simulink model "nonLinearPlant2024"  (R2024a)
settings: Solver=ode45  StartTime=0.0  StopTime=10  RelTol=1e-3
undefined symbols (not defined in the file or in its folder): fractalcoef
libraries: instrumentseriallib x3, simulink x2, instrumentlib x2, mspfiltlib x1, mspsensorlib x1, simulink_extras x1, slpidlib x1
settings Model: LastModifiedBy=saman
settings SolverCC: AutoInsertRateTranBlk=on
settings OptimizationCC: DefaultParameterBehavior=Inlined  EnhancedBackFolding=on  PassReuseOutputArgsAs=Individual arguments  ZeroExternalMemoryAtStartup=off  ZeroInternalMemoryAtStartup=off  MaxStackSize=64  OptimizeBlockOrder=speed  DifferentSizesBufferReuse=on  EfficientTunableParamExpr=on
settings DebuggingCC: ParameterTunabilityLossMsg=error
settings HardwareCC: ProdBitPerPointer=32  ProdBitPerSizeT=32  ProdBitPerPtrDiffT=32  ProdLargestAtomicInteger=Long  ProdLargestAtomicFloat=Double  ProdWordSize=32  ProdHWDeviceType=ARM Compatible->ARM Cortex  UseEmbeddedCoderFeatures=off  UseSimulinkCoderFeatures=off
settings ModelReferenceCC: UpdateModelReferenceTargets=IfOutOfDate
settings SFSimCC: MATLABDynamicMemAlloc=off
settings RTWCC: Description=Embedded Coder  SystemTargetFile=ert.tlc  TemplateMakefile=ert_default_tmf  Toolchain=Arduino ARM  BuildConfiguration=Faster Runs
settings CodeAppCC: ForceParamTrailComments=on  IgnoreCustomStorageClasses=off  OperatorAnnotations=on  SimulinkDataObjDesc=on  SFDataObjDesc=on  InsertBlockDesc=on
settings ERTTargetCC: SupportContinuousTime=on  SupportNonInlinedSFcns=on  ExtModeTransport=3  ExtModeStaticAlloc=on  ExtModeStaticAllocSize=24576  ExtModeMexFile=ext_xcp  ExtModeIntrfLevel=Level2 - Open  InlinedParameterPlacement=NonHierarchical  ERTCustomFileTemplate=example_file_process.tlc

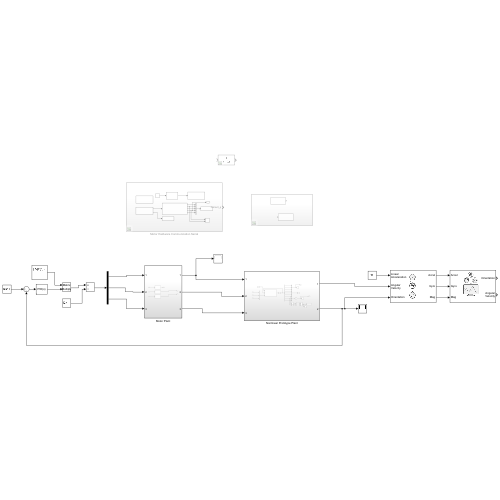
[thumbnail: Simulink's stored preview of the top-level diagram]
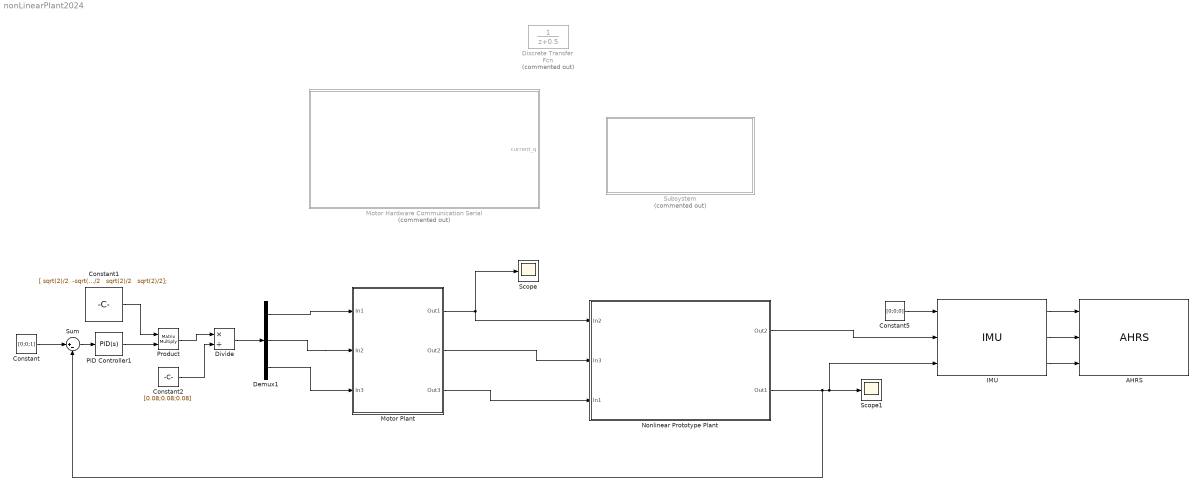
== system nonLinearPlant2024 ==
  AHRS : mspfiltlib/AHRS  DispRefFrame=ENU  DecimationFactor=1  InitialProcessNoise=ahrsfilter.defaultProcessNoise  OrientationFormat=quaternion  SimulateUsing=Interpreted execution  AccelerometerNoise=0.0001924722  GyroscopeNoise=9.1385e-5  MagnetometerNoise=0.1  GyroscopeDriftNoise=3.0462e-13  LinearAccelerationNoise=0.0096236100000000012  MagneticDisturbanceNoise=0.5  LinearAccelerationDecayFactor=0.5  MagneticDisturbanceDecayFactor=0.5  ExpectedMagneticFieldStrength=50
  Constant : Constant  Value=[0;0;1]
  Constant1 : Constant  Value=|
      | [ sqrt(2)/2  -sqrt(2)/4  -sqrt(2)/4;
      |                0           sqrt(6)/4  -sqrt(6)/4;
      |                sqrt(2)/2   sqrt(2)/2   sqrt(2)/2];
  Constant2 : Constant  Value=[0.08;0.08;0.08]
  Constant5 : Constant  Value=[0;0;0]
  Demux1 : Demux  Outputs=3
  Discrete Transfer Fcn : DiscreteTransferFcn  Commented=on
  Divide : Product  Inputs=*/
  IMU : mspsensorlib/IMU  DispRefFrame=ENU  TemperaturePort=off  Temperature=25  MagneticFieldPort=off  MagneticFieldNED=[ 27.5550, -2.4169, -16.0849 ]  MagneticFieldENU=[ -2.4169, 27.5550, 16.0849 ]  SeedDouble=67  SimulateUsing=Interpreted execution  AccelParamsMeasurementRange=Inf  AccelParamsResolution=0  AccelParamsConstantBias=[ 0, 0, 0 ]  AccelParamsAxesMisalignment=[ 100, 0, 0; 0, 100, 0; 0, 0, 100 ]  AccelParamsNoiseDensity=[ 0, 0, 0 ]  AccelParamsBiasInstability=[ 0, 0, 0 ]  AccelParamsBiasInstabilityNumerator=fractalcoef().Numerator  AccelParamsBiasInstabilityDenominator=fractalcoef().Denominator  AccelParamsRandomWalk=[ 0, 0, 0 ]  AccelParamsNoiseType=double-sided  AccelParamsTemperatureBias=[ 0, 0, 0 ]  AccelParamsTemperatureScaleFactor=[ 0, 0, 0 ]  GyroParamsMeasurementRange=Inf  GyroParamsResolution=0  GyroParamsConstantBias=[ 0, 0, 0 ]  GyroParamsAxesMisalignment=[ 100, 0, 0; 0, 100, 0; 0, 0, 100 ]  GyroParamsAccelerationBias=[ 0, 0, 0 ]  GyroParamsNoiseDensity=[ 0, 0, 0 ]  GyroParamsBiasInstability=[ 0, 0, 0 ]  GyroParamsBiasInstabilityNumerator=fractalcoef().Numerator  GyroParamsBiasInstabilityDenominator=fractalcoef().Denominator  GyroParamsRandomWalk=[ 0, 0, 0 ]  GyroParamsNoiseType=double-sided  GyroParamsTemperatureBias=[ 0, 0, 0 ]  GyroParamsTemperatureScaleFactor=[ 0, 0, 0 ]  MagParamsMeasurementRange=Inf  MagParamsResolution=0  MagParamsConstantBias=[ 0, 0, 0 ]  MagParamsAxesMisalignment=[ 100, 0, 0; 0, 100, 0; 0, 0, 100 ]  MagParamsNoiseDensity=[ 0, 0, 0 ]  MagParamsBiasInstability=[ 0, 0, 0 ]  MagParamsBiasInstabilityNumerator=fractalcoef().Numerator  MagParamsBiasInstabilityDenominator=fractalcoef().Denominator  MagParamsRandomWalk=[ 0, 0, 0 ]  MagParamsNoiseType=double-sided  MagParamsTemperatureBias=[ 0, 0, 0 ]  MagParamsTemperatureScaleFactor=[ 0, 0, 0 ]
  Motor Hardware Communication Serial : Subsystem  Commented=on
  Motor Plant : Subsystem
  Nonlinear Prototype Plant : Subsystem
  PID Controller1 : slpidlib/PID Controller  Controller=PID  Form=Parallel  TimeDomain=Continuous-time  UseExternalTs=off  SampleTime=-1  IntegratorMethod=Forward Euler  FilterMethod=Forward Euler  ControllerParametersSource=internal  P=1  I=1  UseKiTs=off  D=0  UseExternalDerivativeSource=off  N=100  UseFilter=on  TunerSelectOption=Transfer Function Based (PID Tuner App)  InitialConditionSource=internal  InitialConditionForIntegrator=0  InitialConditionForFilter=0  DifferentiatorICPrevScaledInput=0  ExternalReset=none  TrackingMode=off  Kt=1  LimitOutput=off  SatLimitsSource=internal  UpperSaturationLimit=inf  LowerSaturationLimit=-inf  LinearizeAsGain=on  AntiWindupMode=none  Kb=1  LimitIntegrator=off  UpperIntegratorSaturationLimit=inf  LowerIntegratorSaturationLimit=-inf  POutMin=[]  POutMax=[]  IOutMin=[]  IOutMax=[]  DOutMin=[]  DOutMax=[]  NOutMin=[]  NOutMax=[]  SumOutMin=[]  SumOutMax=[]  SaturationOutMin=[]  SaturationOutMax=[]  PParamMin=[]  PParamMax=[]  IParamMin=[]  IParamMax=[]  DParamMin=[]  DParamMax=[]  NParamMin=[]  NParamMax=[]  KbParamMin=[]  KbParamMax=[]  KtParamMin=[]  KtParamMax=[]  KbOutMin=[]  KbOutMax=[]  KtOutMin=[]  KtOutMax=[]  IntegratorOutMin=[]  IntegratorOutMax=[]  FilterOutMin=[]  FilterOutMax=[]  SumI1OutMin=[]  SumI1OutMax=[]  SumI2OutMin=[]  SumI2OutMax=[]  SumI3OutMin=[]  SumI3OutMax=[]  SumI4OutMin=[]  SumI4OutMax=[]  SumDOutMin=[]  SumDOutMax=[]  DifferentiatorOutMin=[]  DifferentiatorOutMax=[]  FilterDiffOutCoefMin=[]  FilterDiffOutCoefMax=[]  ReciprocalOutMin=[]  ReciprocalOutMax=[]  SumDenOutMin=[]  SumDenOutMax=[]  SumNumOutMin=[]  SumNumOutMax=[]  DivideOutMin=[]  DivideOutMax=[]  UdiffTsProdOutMin=[]  UdiffTsProdOutMax=[]  NTsProdOutMin=[]  NTsProdOutMax=[]  UintegralTsProdOutMin=[]  UintegralTsProdOutMax=[]  UngainTsProdOutMin=[]  UngainTsProdOutMax=[]  ClampingZeroOutDataTypeStr=Inherit: Inherit via back propagation  ClampingZeroOutMin=[]  ClampingZeroOutMax=[]  FilterDenConstantOutDataTypeStr=Inherit: Inherit via back propagation  FilterDenConstantOutMin=[]  FilterDenConstantOutMax=[]  PCopyOutDataTypeStr=Inherit: Inherit via back propagation  PCopyOutMin=[]  PCopyOutMax=[]  NCopyOutDataTypeStr=Inherit: Inherit via back propagation  NCopyOutMin=[]  NCopyOutMax=[]  IntegratorContinuousStateAttributes=''  IntegratorStateMustResolveToSignalObject=off  IntegratorRTWStateStorageClass=Auto  FilterContinuousStateAttributes=''  FilterStateMustResolveToSignalObject=off  FilterRTWStateStorageClass=Auto  ParallelPVariant=InternalParameters  IdealPVariant=Disabled  IVariant=InternalParameters  DVariant=InternalParameters  IntegratorVariant=Continuous  SatVariant=Disabled  AWVariant=Passthrough  PCopyVariant=Disabled  TRVariant=Disabled  FdbkBlocksVariant=Forward  IdealPFdbkVariant=Disabled  SatFdbkVariant=Disabled  DerivativeFilterVariant=ContFilter  NVariant=InternalParameters  NCopyVariant=Disabled  FilterICVariant=InternalICsFilter  IntegratorICVariant=InternalICs  ExternalResetVariant=Disabled  TRSumVariant=Passthrough  SumFdbkVariant=Disabled  SumVariant=Sum_PID  TsampFilterVariant=InternalTs  TsampNgainVariant=Passthrough  TsampIntegralVariant=Disabled_SignalSpec  ExternalSaturationOutDataTypeStr=Inherit: Same as second input  DerivativeSourceVariant=ErrorSignal
  Product : Product  Multiplication=Matrix(*)
  Scope : Scope
  Scope1 : Scope
  Subsystem : Subsystem  Commented=on
  Sum : Sum  Inputs=|+-
  wires:
  Nonlinear Prototype Plant/2(Out1) -> Sum/2, IMU/3, Scope1/1
  Constant/1 -> Sum/1
  Motor Plant/1(Out1) -> Scope/1, Nonlinear Prototype Plant/1(In2)
  Demux1/2 -> Motor Plant/2(In2)
  Demux1/3 -> Motor Plant/3(In3)
  Motor Plant/2(Out2) -> Nonlinear Prototype Plant/2(In3)
  Motor Plant/3(Out3) -> Nonlinear Prototype Plant/3(In1)
  Product/1 -> Divide/1
  Demux1/1 -> Motor Plant/1(In1)
  Constant1/1 -> Product/1
  Sum/1 -> PID Controller1/1
  PID Controller1/1 -> Product/2
  Divide/1 -> Demux1/1
  Constant2/1 -> Divide/2
  Nonlinear Prototype Plant/1(Out2) -> IMU/2
  Constant5/1 -> IMU/1
  IMU/1 -> AHRS/1
  IMU/2 -> AHRS/2
  IMU/3 -> AHRS/3

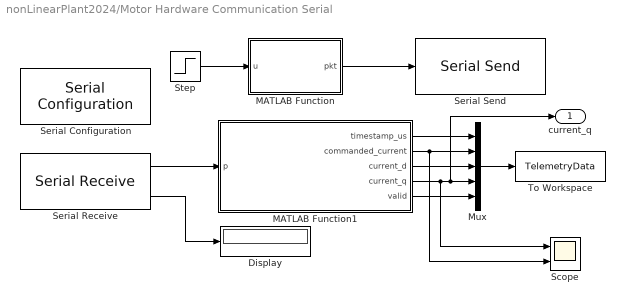
== system nonLinearPlant2024/Motor Hardware Communication Serial ==
  Display : Display
  MATLAB Function : MATLAB Function  TreatAsAtomicUnit=on
  MATLAB Function1 : MATLAB Function  TreatAsAtomicUnit=on
  Mux : Mux  Inputs=5
  Scope : Scope  NumInputPorts=2
  Serial Configuration : instrumentseriallib/Serial Configuration  Priority=-200000  PortSel=COM10  Port=COM10  ComPort=COM10  BaudRate=115200  DataBits=8  Parity=none  StopBits=1  ByteOrder=little-endian  FlowControl=none  Timeout=10  SimulateUsing=Interpreted execution  BlockInModel=on  aMode=1
  Serial Receive : instrumentseriallib/Serial Receive  Priority=1  PortSel=COM10  Port=COM10  ComPort=COM10  DataType=uint8  SaveDataType=uint8  ToggleHeader=on  Header=[165 90]  ToggleDataSize=on  DataSize=[17 1]  ToggleTerminator=on  Terminator=<none>  CustomTerminator=[]  InputFormat=Column major  EnableBlockingMode=off  ActionDataUnavailable=Output last received value  ActionWhenDataUnavailable=Output last received value  CustomValue=0  SampleTime=0.01  SimulateUsing=Interpreted execution  BlockInModel=on  aMode=1
  Serial Send : instrumentseriallib/Serial Send  Priority=1  PortSel=COM10  Port=COM10  ComPort=COM10  Header=[]  Terminator=<none>  CustomTerminator=[]  EnableBlockingMode=off  SimulateUsing=Interpreted execution  BlockInModel=on  aMode=1
  Step : Step  After=0.055  SampleTime=0
  To Workspace : ToWorkspace  VariableName=TelemetryData  SaveFormat=Timeseries  SampleTime=-1
  current_q : Outport
  wires:
  MATLAB Function/1(pkt) -> Serial Send/1
  Step/1 -> MATLAB Function/1(u)
  Serial Receive/1 -> MATLAB Function1/1(p)
  Serial Receive/2 -> Display/1
  MATLAB Function1/1(timestamp_us) -> Mux/1
  MATLAB Function1/2(commanded_current) -> Scope/2, Mux/2
  MATLAB Function1/3(current_d) -> Mux/3
  MATLAB Function1/4(current_q) -> Scope/1, current_q/1, Mux/4
  MATLAB Function1/5(valid) -> Mux/5
  Mux/1 -> To Workspace/1

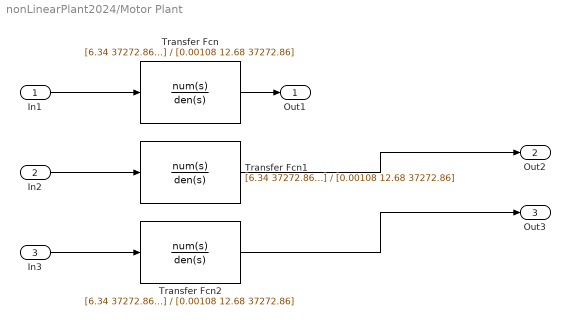
== system nonLinearPlant2024/Motor Plant ==
  In1 : Inport
  In2 : Inport  Port=2
  In3 : Inport  Port=3
  Transfer Fcn : TransferFcn  Numerator=[6.34 37272.86]  Denominator=[0.00108 12.68 37272.86]
  Transfer Fcn1 : TransferFcn  Numerator=[6.34 37272.86]  Denominator=[0.00108 12.68 37272.86]
  Transfer Fcn2 : TransferFcn  Numerator=[6.34 37272.86]  Denominator=[0.00108 12.68 37272.86]
  Out1 : Outport
  Out2 : Outport  Port=2
  Out3 : Outport  Port=3
  wires:
  In1/1 -> Transfer Fcn/1
  Transfer Fcn/1 -> Out1/1
  In3/1 -> Transfer Fcn2/1
  In2/1 -> Transfer Fcn1/1
  Transfer Fcn2/1 -> Out3/1
  Transfer Fcn1/1 -> Out2/1

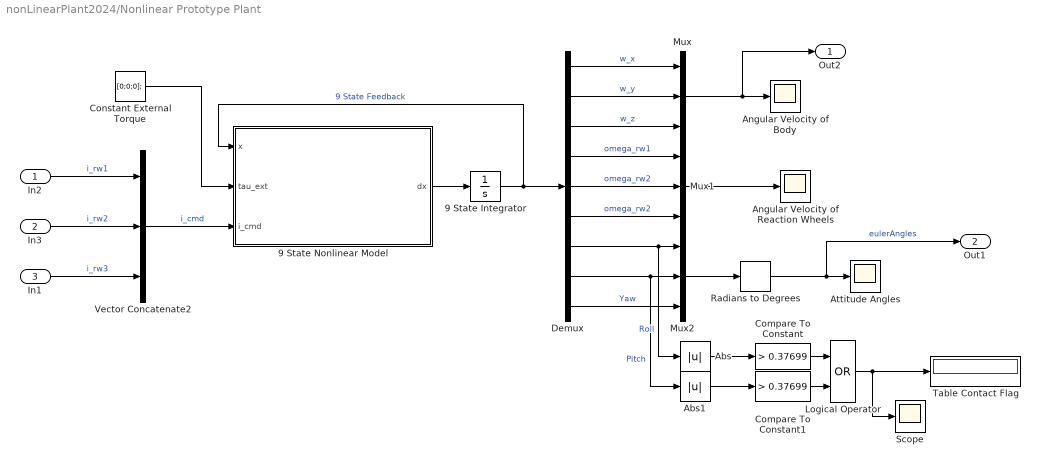
== system nonLinearPlant2024/Nonlinear Prototype Plant ==
  In2 : Inport
  In3 : Inport  Port=2
  In1 : Inport  Port=3
  9 State Integrator : Integrator  InitialCondition=zeros(9,1)  LimitOutput=on  UpperSaturationLimit=[Inf; Inf; Inf; 48.91; 48.91; 48.91; Inf; Inf; Inf];  LowerSaturationLimit=[-Inf; -Inf; -Inf; -48.91; -48.91; -48.91; -Inf; -Inf; -Inf];  ContinuousStateAttributes={'wX','wY','wZ','omegaX','omegaY','omegaZ','roll','pitch','yaw'}
  9 State Nonlinear Model : MATLAB Function  TreatAsAtomicUnit=on
  Abs : Abs  SaturateOnIntegerOverflow=off
  Abs1 : Abs  SaturateOnIntegerOverflow=off
  Angular Velocity of Body : Scope
  Angular Velocity of Reaction Wheels : Scope
  Attitude Angles : Scope
  Compare To Constant : simulink/Logic and Bit Operations/Compare To Constant  relop=>  const=0.37699  OutDataTypeStr=boolean
  Compare To Constant1 : simulink/Logic and Bit Operations/Compare To Constant  relop=>  const=0.37699  OutDataTypeStr=boolean
  Constant External Torque : Constant  Value=[0;0;0];
  Demux : Demux  Outputs=9
  Logical Operator : Logic  Operator=OR  AllPortsSameDT=off  OutDataTypeStr=boolean
  Mux : Mux  Inputs=3
  Mux1 : Mux  Inputs=3
  Mux2 : Mux  Inputs=3
  Radians to Degrees : simulink_extras/Transformations/Radians to Degrees
  Scope : Scope
  Table Contact Flag : Display
  Vector Concatenate2 : Concatenate  NumInputs=3
  Out2 : Outport
  Out1 : Outport  Port=2
  wires:
  Demux/5 -> Mux1/2  "omega_rw2"
  Compare To Constant/1 -> Logical Operator/1
  9 State Integrator/1 -> 9 State Nonlinear Model/1(x), Demux/1  "9 State Feedback"
  Demux/7 -> Abs/1, Mux2/1  "Roll"
  Demux/1 -> Mux/1  "w_x"
  Demux/4 -> Mux1/1  "omega_rw1"
  Demux/9 -> Mux2/3  "Yaw"
  Mux/1 -> Out2/1, Angular Velocity of Body/1
  Demux/3 -> Mux/3  "w_z"
  Constant External Torque/1 -> 9 State Nonlinear Model/2(tau_ext)
  Compare To Constant1/1 -> Logical Operator/2
  Demux/8 -> Abs1/1, Mux2/2  "Pitch"
  Abs1/1 -> Compare To Constant1/1
  Mux1/1 -> Angular Velocity of Reaction Wheels/1
  Demux/2 -> Mux/2  "w_y"
  Mux2/1 -> Radians to Degrees/1
  Abs/1 -> Compare To Constant/1
  9 State Nonlinear Model/1(dx) -> 9 State Integrator/1
  Vector Concatenate2/1 -> 9 State Nonlinear Model/3(i_cmd)  "i_cmd"
  Demux/6 -> Mux1/3  "omega_rw2"
  Radians to Degrees/1 -> Out1/1, Attitude Angles/1  "eulerAngles"
  Logical Operator/1 -> Scope/1, Table Contact Flag/1
  In1/1 -> Vector Concatenate2/3  "i_rw3"
  In3/1 -> Vector Concatenate2/2  "i_rw2"
  In2/1 -> Vector Concatenate2/1  "i_rw1"

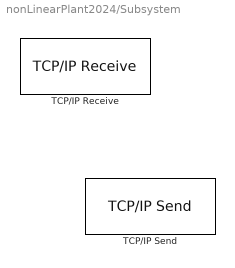
== system nonLinearPlant2024/Subsystem ==
  TCP/IP Receive : instrumentlib/TCP//IP Receive  Port=80  DataSize=[ 1, 1 ]  DataType=uint8  ASCIIFormatting=%f  Terminator=LF  CustomTerminator=10  ByteOrder=big-endian  EnableBlockingMode=on  Timeout=10  SampleTime=0.01  SimulateUsing=Interpreted execution
  TCP/IP Send : instrumentlib/TCP//IP Send  Port=80  ByteOrder=big-endian  EnableBlockingMode=on  Timeout=10  TransferDelay=on  SimulateUsing=Interpreted execution

== matlab function nonLinearPlant2024/Motor Hardware Communication Serial/MATLAB Function1 ==
  data: p input; timestamp_us output; commanded_current output; current_d output; current_q output; valid output
function [timestamp_us, commanded_current, current_d, current_q, valid] = UnpackTelemetry(p)
   
    % Input: 17 bytes after the A5 5A header
    % Payload: timestamp (uint32), commanded current, Id, Iq, checksum
    
    b = reshape(uint8(p), 1, 17);
    
    % Verify XOR checksum over timestamp and three current values
    cs = uint8(0);
    for k = 1:16
        cs = bitxor(cs, b(k));
    end
    
    valid = (cs == b(17));
    
    % Decode binary data
    timestamp_us = typecast(uint8(b(1:4)), 'uint32');
    commanded_current = typecast(uint8(b(5:8)), 'single');
    current_d = typecast(uint8(b(9:12)), 'single');
    current_q = typecast(uint8(b(13:16)), 'single');
    
    % Reject invalid current measurements
    if ~valid
        commanded_current = single(NaN);
        current_d = single(NaN);
        current_q = single(NaN);
    end
end

== matlab function nonLinearPlant2024/Motor Hardware Communication Serial/MATLAB Function ==
  data: u input; pkt output
function pkt = PackCommand(u)

    u = single(u);
    b = reshape(typecast(u, 'uint8'), 1, 4);
    
    pkt = zeros(1, 7, 'uint8');
    
    pkt(1) = uint8( hex2dec('A5') );
    pkt(2) = uint8( hex2dec('5A') );
    pkt(3:6) = b;
    
    cs = uint8(0);
    for k = 3:6
        cs = bitxor(cs, pkt(k));
    end
    
    pkt(7) = cs;
end

== matlab function nonLinearPlant2024/Nonlinear Prototype Plant/9 State Nonlinear Model ==
  data: x input; dx output; tau_ext input; i_cmd input
function dx = nonlinearPlant(x,tau_ext,i_cmd)
    
    % Protoype system inertia matrix
    I = [0.250909017 0 0;
         0 0.25037717 0;
         0 0 0.449674125];
    
    % RW inertia matrix
    I_rw = [0.000637038 0 0; 
            0 0.000637038 0;
            0 0 0.000637038];

    % Torque constant of rw, [Nm/A]
    kt_rw1 = 0.08; 
    kt_rw2 = 0.08;
    kt_rw3 = 0.08;

% Reaction wheel frame to body frame
    R_b_rw = [ sqrt(2)/2  -sqrt(2)/4  -sqrt(2)/4;
               0           sqrt(6)/4  -sqrt(6)/4;
               sqrt(2)/2   sqrt(2)/2   sqrt(2)/2];
    
    
    % Initiate states and vectors
    wx = x(1);
    wy = x(2);
    wz = x(3);
    
    Omega_x = x(4);
    Omega_y = x(5);
    Omega_z = x(6);
    
    phi   = x(7);
    theta = x(8);
    psi   = x(9);
    
    w = [wx;wy;wz];

    Omega = [Omega_x;Omega_y;Omega_z];

    % Reaction wheel input is current
    kt_rw = [kt_rw1;
             kt_rw2;
             kt_rw3];
 
    tau_rw = kt_rw .* i_cmd;

    Omega_dot = I_rw \ tau_rw;


    % Dynamic equation for prototype
    w_dot = I \ ( ...
        tau_ext ...
        - cross(w,I*w) ...
        - R_b_rw*(I_rw*Omega_dot) ...
        - cross(w,R_b_rw*(I_rw*Omega)) );

   % Euler kinematics
    phi_dot = ...
        wx ...
        + wy*sin(phi)*tan(theta) ...
        + wz*cos(phi)*tan(theta);
    
    theta_dot = ...
        wy*cos(phi) ...
        - wz*sin(phi);
    
    psi_dot = ...
        (wy*sin(phi) ...
        + wz*cos(phi)) / cos(theta);
    
    % State derivatives of system
    dx = [
        w_dot;
        Omega_dot;
        phi_dot;
        theta_dot;
        psi_dot
    ];
end
